simulink model "Slope_Road_SideSlipAngle_Vx_Estimation"  (R2024b)
settings: Solver=FixedStepAuto  StartTime=0.0  StopTime=7.5  FixedStep=0.001  RelTol=1e-4
values from neighbouring files (symbols this model uses):
  ax_long_1 = 1    [Init.m]
  ax_long_2 = 3    [Init.m]
  ax_long_3 = 6    [Init.m]
  ax_steer_1 = 0.5    [Init.m]
  ax_steer_2 = 1.5    [Init.m]
  ax_steer_3 = 3    [Init.m]
  ax_vx_thres1 = 0.5    [Init.m]
  ax_vx_thres2 = 3    [Init.m]
  Brush = [28.93,1.496,0.9486,0.06054]    [Init.m]
  delay_constant = 1/delay_length*ones(1,round(delay_length))    [Init.m]
  delta_thres = 3*3.14/180    (= 0.0523333333333)    [Init.m]
  deltarate_thres = 0.1    [Init.m]
  dg2rd = pi/180    (= 0.0174532925199)    [Init.m]
  excessive_wheel_intgr = 1000    [Init.m]
  filter_ratio_ax_ay = 0.2    [Init.m]
  g = 9.8    [Init.m]
  gao_ay = 1.5    [Init.m]
  gao_D_v = 0.2    [Init.m]
  gao_D_w = 0.03    [Init.m]
  gao_D_w1 = 0.25    [Init.m]
  gao_gz = 0.1    [Init.m]
  gao_Q = 1e-02    (= 0.01)    [Init.m]
  gao_R = 0.00077574*0.1    (= 7.7574e-05)    [Init.m]
  K_theta = 1    [Init.m]
  k_vx_vari_thres1 = 20    [Init.m]
  k_vx_vari_thres2 = 20    [Init.m]
  k_vx_vari_thres3 = 20    [Init.m]
  k_vy = 1/veh_m0    (= 0.000327653997379)    [Init.m]
  N_num = 6    [Init.m]
  para_long_1 = 1    [Init.m]
  para_long_2 = 100    [Init.m]
  para_long_3 = 100000000    [Init.m]
  para_long_4 = 100    [Init.m]
  para_steer_1 = 0.1    [Init.m]
  para_steer_2 = 10    [Init.m]
  para_steer_3 = 1000    [Init.m]
  para_steer_4 = 1000    [Init.m]
  rd2dg = 180/pi    (= 57.2957795131)    [Init.m]
  Steer_angle = 0    [Init.m]
  tao_1 = 6    [Init.m]
  time_interval = 1/Ts    (= 1000)    [Init.m]
  Ts = 0.001    [Init.m]
  u_init = 0.9    [Init.m]
  veh_bf = 1.600    (= 1.6)    [Init.m]
  veh_br = 1.740    (= 1.74)    [Init.m]
  veh_lf = 1.293    [Init.m]
  veh_lr = veh_l-veh_lf    (= 1.835)    [Init.m]
  veh_m0 = 3052    [Init.m]
  vx_cri = 1    [Init.m]
  vx_lowest = 0.01    [Init.m]
  vx_max_diff = 1    [Init.m]
  vy_new_ini = 0    [Init.m]
  wh_r = 0.346    [Init.m]
undefined symbols (not defined in the file or in its folder): DiscIntNeverNeededParam, front_gear_ratio, rear_gear_ratio, steer_ratio
libraries: simulink x7, Solver_SF x1
(part 2 of 2)

== system Slope_Road_SideSlipAngle_Vx_Estimation/vx estimation/detect overslip // excessive wheel slip(ews)/wheel acceleration deviation criterion/车轮加速度2/Subsystem1 ==
  In1 : Inport
  Mux : Mux  Inputs=10
  Unit Delay{1..9} (9 alike) : UnitDelay  SampleTime=-1  HasFrameUpgradeWarning=on
  last : Outport
  Out1 : Outport  Port=2
  wires:
  Mux/1 -> Out1/1
  In1/1 -> Mux/10, Unit Delay3/1
  Unit Delay9/1 -> last/1, Mux/1
  Unit Delay8/1 -> Mux/2, Unit Delay9/1
  Unit Delay7/1 -> Mux/3, Unit Delay8/1
  Unit Delay6/1 -> Mux/4, Unit Delay7/1
  Unit Delay5/1 -> Mux/5, Unit Delay6/1
  Unit Delay4/1 -> Mux/6, Unit Delay5/1
  Unit Delay1/1 -> Mux/8, Unit Delay2/1
  Unit Delay2/1 -> Mux/7, Unit Delay4/1
  Unit Delay3/1 -> Mux/9, Unit Delay1/1

== system Slope_Road_SideSlipAngle_Vx_Estimation/vx estimation/detect overslip // excessive wheel slip(ews)/wheel acceleration deviation criterion/车轮加速度2/Subsystem2 ==
  In1 : Inport
  Mux : Mux  Inputs=10
  Unit Delay{1..9} (9 alike) : UnitDelay  SampleTime=-1  HasFrameUpgradeWarning=on
  last : Outport
  Out1 : Outport  Port=2
  wires:
  Unit Delay3/1 -> Mux/9, Unit Delay1/1
  Unit Delay2/1 -> Mux/7, Unit Delay4/1
  Unit Delay1/1 -> Mux/8, Unit Delay2/1
  Unit Delay4/1 -> Mux/6, Unit Delay5/1
  Unit Delay5/1 -> Mux/5, Unit Delay6/1
  Unit Delay6/1 -> Mux/4, Unit Delay7/1
  Unit Delay7/1 -> Mux/3, Unit Delay8/1
  Unit Delay8/1 -> Mux/2, Unit Delay9/1
  Unit Delay9/1 -> Mux/1, last/1
  In1/1 -> Mux/10, Unit Delay3/1
  Mux/1 -> Out1/1

== system Slope_Road_SideSlipAngle_Vx_Estimation/vx estimation/detect overslip // excessive wheel slip(ews)/wheel acceleration deviation criterion/车轮加速度3/Subsystem ==
  In1 : Inport
  Mux : Mux  Inputs=10
  Unit Delay{,1..8} (9 alike) : UnitDelay  SampleTime=-1  HasFrameUpgradeWarning=on
  last : Outport
  Out1 : Outport  Port=2
  wires:
  Mux/1 -> Out1/1
  In1/1 -> Unit Delay/1, Mux/10
  Unit Delay8/1 -> last/1, Mux/1
  Unit Delay7/1 -> Unit Delay8/1, Mux/2
  Unit Delay6/1 -> Unit Delay7/1, Mux/3
  Unit Delay5/1 -> Unit Delay6/1, Mux/4
  Unit Delay4/1 -> Unit Delay5/1, Mux/5
  Unit Delay3/1 -> Unit Delay4/1, Mux/6
  Unit Delay1/1 -> Unit Delay2/1, Mux/8
  Unit Delay2/1 -> Unit Delay3/1, Mux/7
  Unit Delay/1 -> Unit Delay1/1, Mux/9

== system Slope_Road_SideSlipAngle_Vx_Estimation/vx estimation/detect overslip // excessive wheel slip(ews)/wheel acceleration deviation criterion/车轮加速度3/Subsystem1 ==
  In1 : Inport
  Mux : Mux  Inputs=10
  Unit Delay{1..9} (9 alike) : UnitDelay  SampleTime=-1  HasFrameUpgradeWarning=on
  last : Outport
  Out1 : Outport  Port=2
  wires:
  Unit Delay3/1 -> Unit Delay1/1, Mux/9
  Unit Delay2/1 -> Unit Delay4/1, Mux/7
  Unit Delay1/1 -> Unit Delay2/1, Mux/8
  Unit Delay4/1 -> Unit Delay5/1, Mux/6
  Unit Delay5/1 -> Unit Delay6/1, Mux/5
  Unit Delay6/1 -> Unit Delay7/1, Mux/4
  Unit Delay7/1 -> Unit Delay8/1, Mux/3
  Unit Delay8/1 -> Unit Delay9/1, Mux/2
  Unit Delay9/1 -> Mux/1, last/1
  In1/1 -> Unit Delay3/1, Mux/10
  Mux/1 -> Out1/1

== system Slope_Road_SideSlipAngle_Vx_Estimation/vx estimation/detect overslip // excessive wheel slip(ews)/wheel acceleration deviation criterion/车轮加速度3/Subsystem2 ==
  In1 : Inport
  Mux : Mux  Inputs=10
  Unit Delay{1..9} (9 alike) : UnitDelay  SampleTime=-1  HasFrameUpgradeWarning=on
  last : Outport
  Out1 : Outport  Port=2
  wires:
  Mux/1 -> Out1/1
  In1/1 -> Unit Delay3/1, Mux/10
  Unit Delay9/1 -> last/1, Mux/1
  Unit Delay8/1 -> Unit Delay9/1, Mux/2
  Unit Delay7/1 -> Unit Delay8/1, Mux/3
  Unit Delay6/1 -> Unit Delay7/1, Mux/4
  Unit Delay5/1 -> Unit Delay6/1, Mux/5
  Unit Delay4/1 -> Unit Delay5/1, Mux/6
  Unit Delay1/1 -> Unit Delay2/1, Mux/8
  Unit Delay2/1 -> Unit Delay4/1, Mux/7
  Unit Delay3/1 -> Unit Delay1/1, Mux/9

== system Slope_Road_SideSlipAngle_Vx_Estimation/vx estimation/detect overslip // excessive wheel slip(ews)/wheel acceleration deviation criterion/车轮加速度4/Subsystem ==
  In1 : Inport
  Mux : Mux  Inputs=10
  Unit Delay{,1..8} (9 alike) : UnitDelay  SampleTime=-1  HasFrameUpgradeWarning=on
  last : Outport
  Out1 : Outport  Port=2
  wires:
  Unit Delay/1 -> Mux/9, Unit Delay1/1
  Unit Delay2/1 -> Mux/7, Unit Delay3/1
  Unit Delay1/1 -> Mux/8, Unit Delay2/1
  Unit Delay3/1 -> Mux/6, Unit Delay4/1
  Unit Delay4/1 -> Mux/5, Unit Delay5/1
  Unit Delay5/1 -> Mux/4, Unit Delay6/1
  Unit Delay6/1 -> Mux/3, Unit Delay7/1
  Unit Delay7/1 -> Mux/2, Unit Delay8/1
  Unit Delay8/1 -> Mux/1, last/1
  In1/1 -> Mux/10, Unit Delay/1
  Mux/1 -> Out1/1

== system Slope_Road_SideSlipAngle_Vx_Estimation/vx estimation/detect overslip // excessive wheel slip(ews)/wheel acceleration deviation criterion/车轮加速度4/Subsystem1 ==
  In1 : Inport
  Mux : Mux  Inputs=10
  Unit Delay{1..9} (9 alike) : UnitDelay  SampleTime=-1  HasFrameUpgradeWarning=on
  last : Outport
  Out1 : Outport  Port=2
  wires:
  Mux/1 -> Out1/1
  In1/1 -> Mux/10, Unit Delay3/1
  Unit Delay9/1 -> last/1, Mux/1
  Unit Delay8/1 -> Mux/2, Unit Delay9/1
  Unit Delay7/1 -> Mux/3, Unit Delay8/1
  Unit Delay6/1 -> Mux/4, Unit Delay7/1
  Unit Delay5/1 -> Mux/5, Unit Delay6/1
  Unit Delay4/1 -> Mux/6, Unit Delay5/1
  Unit Delay1/1 -> Mux/8, Unit Delay2/1
  Unit Delay2/1 -> Mux/7, Unit Delay4/1
  Unit Delay3/1 -> Mux/9, Unit Delay1/1

== system Slope_Road_SideSlipAngle_Vx_Estimation/vx estimation/detect overslip // excessive wheel slip(ews)/wheel acceleration deviation criterion/车轮加速度4/Subsystem2 ==
  In1 : Inport
  Mux : Mux  Inputs=10
  Unit Delay{1..9} (9 alike) : UnitDelay  SampleTime=-1  HasFrameUpgradeWarning=on
  last : Outport
  Out1 : Outport  Port=2
  wires:
  Unit Delay3/1 -> Mux/9, Unit Delay1/1
  Unit Delay2/1 -> Mux/7, Unit Delay4/1
  Unit Delay1/1 -> Mux/8, Unit Delay2/1
  Unit Delay4/1 -> Mux/6, Unit Delay5/1
  Unit Delay5/1 -> Mux/5, Unit Delay6/1
  Unit Delay6/1 -> Mux/4, Unit Delay7/1
  Unit Delay7/1 -> Mux/3, Unit Delay8/1
  Unit Delay8/1 -> Mux/2, Unit Delay9/1
  Unit Delay9/1 -> Mux/1, last/1
  In1/1 -> Mux/10, Unit Delay3/1
  Mux/1 -> Out1/1

== matlab function Slope_Road_SideSlipAngle_Vx_Estimation/side slip angle estimation /side slip angle estimation/MATLAB Function ==
  data: delta input; m input; vx input; omega input; ay input; vy_hat_deri output; excita input; theta_hat input; fy_hat_star input; par_fystar_vy input; k_vy input; tao_1 input; Fx_front input; time_sig input; time_sig output; K_theta input; time_interval input; ema output; ota output
function [vy_hat_deri, time_sig,ema,ota] = fcn(delta, m, vx, omega, ay, excita, theta_hat, fy_hat_star,par_fystar_vy,k_vy, tao_1, Fx_front, time_sig, K_theta, time_interval)

if abs(m*ay)<abs(theta_hat*fy_hat_star) && par_fystar_vy>-abs(fy_hat_star)
    ema=-abs(fy_hat_star);
    ota=1/(2*max(abs(fy_hat_star),0.01));
else
    ema=par_fystar_vy;
    ota=1/max((ema^2+fy_hat_star^2)^(0.5),0.01);
end

%  vy_hat_deri=ay-omega*vx+k_vy*ota*ema*(m*ay-Fx_front*sin(delta)-theta_hat*fy_hat_star);  % 估计器公式
% vy_hat_deri=ay-omega*vx+k_vy*ota*ema*(m*ay-Fx_front*sin(delta)-fy_hat_star);  % 估计器公式
vy_hat_deri=ay-omega*vx+k_vy*ota*ema*(m*ay-fy_hat_star);  % 估计器公式



%  if excita==1  % 激励充足
% %      theta_hat_deri=tao_1*k_vy*ota*fy_hat_star*(m*ay-Fx_front*sin(delta)-theta_hat*fy_hat_star);  % 估计器公式
%      theta_hat_deri=tao_1*k_vy*ota*fy_hat_star*(m*ay-Fx_front*sin(delta)-fy_hat_star);  % 估计器公式
%      time_sig=0;
%  else          % 激励不足
%      time_sig=time_sig+1;
%      if time_sig>=time_interval    % 激励不足持续一段时间
%         theta_hat_deri=K_theta*(1-theta_hat) ;   % theta逐渐收敛到1
%      else
%         theta_hat_deri=0;     % theta不更新
%      end     
%  end

== matlab function Slope_Road_SideSlipAngle_Vx_Estimation/side slip angle estimation /MATLAB Function2 ==
  data: vx input; y output; vx_cri input
function y = fcn(vx,vx_cri)

if vx<=vx_cri
    y=vx_cri;
else
    y=vx;
end

== matlab function Slope_Road_SideSlipAngle_Vx_Estimation/vx estimation/Kalman-Filter/Kalman Gain/MATLAB Function ==
  data: ews input; R_update output; ax_pro input; vbest_believe input; gao_R input; gao_Q input; Q_update output; para_long_1 input; para_long_2 input; para_long_3 input; para_long_4 input; para_steer_1 input; para_steer_2 input; para_steer_3 input; para_steer_4 input; ax_long_1 input; ax_long_2 input; ax_long_3 input; ax_steer_1 input; ax_steer_2 input; ax_steer_3 input
function [R_update,Q_update] = fcn(ews, ax_pro, vbest_believe,gao_R,gao_Q,para_long_1,para_long_2,para_long_3,para_long_4,para_steer_1,para_steer_2,para_steer_3,para_steer_4,ax_long_1,ax_long_2,ax_long_3,ax_steer_1,ax_steer_2,ax_steer_3)
if  vbest_believe==0  % 没有侧向运动
   if ((sum(ews)>=0 & sum(ews)<=2) || abs(ax_pro)<=ax_long_1) && (abs(ax_pro)<=ax_long_2)
        R_update=para_long_1*gao_R;
        Q_update=gao_Q;
   elseif ((sum(ews)==3) || (abs(ax_pro)<=ax_long_2 & abs(ax_pro)>ax_long_1)) && (abs(ax_pro)<=ax_long_3)
        rate_long_1=(para_long_2-para_long_1)/(ax_long_2-ax_long_1);
        R_update=(para_long_1+rate_long_1*(abs(ax_pro)-ax_long_1))*gao_R;
        Q_update=gao_Q;
   else
        rate_long_2=(para_long_3-para_long_2)/(ax_long_3-ax_long_2);
        R_update=(para_long_2+rate_long_2*(abs(ax_pro)-ax_long_2))*gao_R;
        Q_update=para_long_4*gao_Q;
   end
else
   if (sum(ews)>=0 & sum(ews)<=2) || abs(ax_pro)<=ax_steer_1
        R_update=para_steer_1*gao_R;
        Q_update=gao_Q;
   elseif (sum(ews)==3) || (abs(ax_pro)<=ax_steer_2 & abs(ax_pro)>ax_steer_1)
        rate_steer_1=(para_steer_2-para_steer_1)/(ax_steer_2-ax_steer_1);
        R_update=(para_steer_1+rate_steer_1*(abs(ax_pro)-ax_steer_1))*gao_R;
        Q_update=gao_Q;
   else
        rate_steer_2=(para_steer_3-para_steer_2)/(ax_steer_3-ax_steer_2);
        R_update=(para_steer_2+rate_steer_2*(abs(ax_pro)-ax_steer_2))*gao_R;
        Q_update=para_steer_4*gao_Q;
   end
end

== matlab function Slope_Road_SideSlipAngle_Vx_Estimation/vx estimation/best wheel selection /MATLAB Function3 ==
  data: v output size=[1,1]; vrc input; ews input; ay input; gao_ay input; gz input; gao_gz input; Fxfl_sign input; Fxfr_sign input; Fxrl_sign input; Fxrr_sign input; v_best_believe output size=[1,1]; delta_rad input; deltarate_rads input; delta_thres input; deltarate_thres input
function [v,v_best_believe] = fcn(vrc,ews,ay,gao_ay,gz,gao_gz,Fxfl_sign,Fxfr_sign,Fxrl_sign,Fxrr_sign,delta_rad,deltarate_rads,delta_thres,deltarate_thres)


vFL = vrc(1);   % v_corr FL
vFR = vrc(2);   % v_corr FR
vRL = vrc(3);   % v_corr RL
vRR = vrc(4);   % v_corr RR
ewsFL = ews(1); % ews FL
ewsFR = ews(2); % ews FR
ewsRL = ews(3); % ews RL
ewsRR = ews(4); % ews RR
v=zeros(1,1);
v_choose_p=zeros(4,2);
v_choose_l=zeros(4,2);
v_choose = [ewsFL vFL Fxfl_sign; 
            ewsFR vFR Fxfr_sign; 
            ewsRL vRL Fxrl_sign; 
            ewsRR vRR Fxrr_sign]; % All velocities with corresponding EWS Flag
v_best_believe=boolean(1);

%我们发现，纵向加速度的测量值会受到坡度的影响，因此有时纵向加速度为正，实际车辆在减速，容易影响最优车速的选择；此外横摆角速度和侧向车速也会影响纵向加速度。因此我们采用每个车轮上是否有加速或减速意图（通过轮胎上施加的是驱动力还是制动力来判断）来判断某个轮胎处于驱动还是制动状态。
if ((abs(ay)>=gao_ay | abs(gz)>gao_gz | abs(delta_rad)>delta_thres | abs(deltarate_rads)>deltarate_thres) )  
    % 有侧向运动的情况
     if sum(ews(1:4)) == 4   % If all wheels have EWS, choose from all 4 wheels
        v_choose_f1 = [vFL Fxfl_sign; vFR Fxfr_sign; vRL Fxrl_sign; vRR Fxrr_sign];
        v=all_wheel_slip(v_choose_f1(:,1),sum(v_choose_f1(:,2)));
     else
        lenth_l=sum(v_choose(:,1)==0);  % 不打滑车轮数量
        num_index_l=(v_choose(:,1)==0);  % 车轮打滑为0，不打滑为1
        jj=0;
        for ii=1:4
            if num_index_l(ii)==1
                jj=jj+1;
                v_choose_l(jj,:)=v_choose(ii,2:3);  % 筛选不打滑车轮的信息
            end
        end
        if lenth_l==4  % 四轮不打滑
             v=all_wheel_slip_lat(v_choose_l(1:lenth_l,1),lenth_l);
        elseif lenth_l==3  % 三轮不打滑
             v=all_wheel_slip_lat(v_choose_l(1:lenth_l,1),lenth_l);
        else
             v=mean(v_choose_l(1:lenth_l,1));
        end
    end
    v_best_believe=boolean(1);
else
    if sum(ews(1:4)) == 4   % If all wheels have EWS, choose from all 4 wheels
        v_choose_f2 = [vFL Fxfl_sign; vFR Fxfr_sign; vRL Fxrl_sign; vRR Fxrr_sign];
        v=all_wheel_slip(v_choose_f2(:,1),sum(v_choose_f2(:,2)));  %取最小或最大轮速
    else
        lenth=sum(v_choose(:,1)==0);
        num_index=(v_choose(:,1)==0);
        j=0;
        for i=1:4
            if num_index(i)==1
                j=j+1;
                v_choose_p(j,:)=v_choose(i,2:3);  % 筛选不打滑车轮的信息
            end
        end
        if (sum(v_choose_p(:,2)>0)==lenth)  % 不打滑车轮的纵向力均为正
           v=min(v_choose_p(1:lenth,1));
        elseif (sum(v_choose_p(:,2)<0)==lenth)  % 不打滑车轮的纵向力均为负
           v=max(v_choose_p(1:lenth,1)); 
        else   % 不打滑车轮的纵向力正负不统一
           v=all_wheel_slip_long(v_choose_p(:,1),lenth);  
        end
    end
  v_best_believe=boolean(0);
end
end

== matlab function Slope_Road_SideSlipAngle_Vx_Estimation/vx estimation/detect overslip // excessive wheel slip(ews)/MATLAB Function ==
  data: u1 input; y output; u2 input; vr input; excessive_wheel_intgr input; intgr_num_pre input; intgr_num output; vx_max_diff input
function [y, intgr_num] = fcn(u1,u2,vr,excessive_wheel_intgr,intgr_num_pre,vx_max_diff)

num=length(u2);
y=zeros(num,1);
vx_ave=mean(vr);
vx_diff=max(abs(vr-vx_ave));
intgr_num=zeros(num,1);
for i=1:num
    if u1(i)>=1 
        y(i)=u1(i)+u2(i);
        intgr_num(i)=0;
    elseif u1(i)<1 & intgr_num_pre(i)<=excessive_wheel_intgr(i)
        if vx_diff>=vx_max_diff
            y(i)=u1(i)+u2(i);
            intgr_num(i)=0;
        else
            y(i)=u1(i)+u2(i);
            intgr_num(i)=intgr_num_pre(i)+1;  % 若u1=0，四轮轮速差异不大，计时1s（或0.1s），在1s内信任u2，1s后不信任u2
        end
    else
        y(i)=u1(i);%+u2(i);
        intgr_num(i)=0;
    end
end

== matlab function Slope_Road_SideSlipAngle_Vx_Estimation/vx estimation/detect overslip // excessive wheel slip(ews)/pre estimation deviation criterion/Embedded MATLAB Function ==
  data: u input; y output; gao_D_v input
function y = fcn(u,gao_D_v)
%#eml



p=size(u);
if p(1)~=4 | p(2)~=1
    y=zeros(4,1);
    y=gao_D_v+0.01;
else
         y=u;
end

== matlab function Slope_Road_SideSlipAngle_Vx_Estimation/vx estimation/detect overslip // excessive wheel slip(ews)/wheel acceleration deviation criterion/Embedded MATLAB Function ==
  data: u input; y output; gao_D_w1 input; p output
function [y,p] = fcn(u,gao_D_w1)
%#eml

p=size(u);
if p(1)~=4 | p(2)~=1
    y=zeros(4,1);
    y=gao_D_w1+0.01;
else
         y=u;

end

== matlab function Slope_Road_SideSlipAngle_Vx_Estimation/vx estimation/detect overslip // excessive wheel slip(ews)/wheel acceleration deviation criterion/车轮加速度1/Embedded MATLAB Function ==
  data: y input; a output; N input
function a = fcn(y, N)
%#eml
ak=single(0);
 k=single(length(y));
for n=0:N-1
h= 6/(N*(N+1))*(1-2*n/(N-1));
ak=ak+h*y(k-n);
end
a = ak;

== matlab function Slope_Road_SideSlipAngle_Vx_Estimation/vx estimation/detect overslip // excessive wheel slip(ews)/wheel acceleration deviation criterion/车轮加速度2/Embedded MATLAB Function ==
  data: y input; a output; N input; m output
function [a,m] = fcn(y, N)
%#eml
ak=single(0);
 k=single(length(y));
for n=0:N-1
h= 6/(N*(N+1))*(1-2*n/(N-1));
ak=ak+h*y(k-n);
end
a = ak;
m=length(y);

== matlab function Slope_Road_SideSlipAngle_Vx_Estimation/vx estimation/detect overslip // excessive wheel slip(ews)/wheel acceleration deviation criterion/车轮加速度3/Embedded MATLAB Function ==
  data: y input; a output; N input
function a = fcn(y, N)
%#eml
ak=single(0);
 k=single(length(y));
for n=0:N-1
h= 6/(N*(N+1))*(1-2*n/(N-1));
ak=ak+h*y(k-n);
end
a = ak;

== matlab function Slope_Road_SideSlipAngle_Vx_Estimation/vx estimation/detect overslip // excessive wheel slip(ews)/wheel acceleration deviation criterion/车轮加速度4/Embedded MATLAB Function ==
  data: y input; a output; N input
function a = fcn(y, N)
%#eml
ak=single(0);
 k=single(length(y));
for n=0:N-1
h= 6/(N*(N+1))*(1-2*n/(N-1));
ak=ak+h*y(k-n);
end
a = ak;

== matlab function Slope_Road_SideSlipAngle_Vx_Estimation/vx estimation/detect overslip // excessive wheel slip(ews)/wheel speed change criterion/Embedded MATLAB Function ==
  data: u input; y output; gao_D_w input
function y = fcn(u,gao_D_w)
%#eml
p=size(u);
if p(1)~=4 | p(2)~=1
    y=zeros(4,1);
    y=gao_D_w+0.01;
else
         y=u;
end

== matlab function Slope_Road_SideSlipAngle_Vx_Estimation/vx estimation/front_rear_drive process/Atomic Subsystem/MATLAB Function ==
  data: ax input; y output; ax_vx_thres1 input; ax_vx_thres2 input; k_vx_vari_thres1 input; k_vx_vari_thres2 input; k_vx_vari_thres3 input
function y = fcn(ax,ax_vx_thres1,ax_vx_thres2,k_vx_vari_thres1,k_vx_vari_thres2,k_vx_vari_thres3)
if abs(ax)<=ax_vx_thres1
    y=k_vx_vari_thres1;
elseif abs(ax)>ax_vx_thres1 & abs(ax)<=ax_vx_thres2
     y=k_vx_vari_thres2;
else
y=k_vx_vari_thres3;
end

== matlab function Slope_Road_SideSlipAngle_Vx_Estimation/vx estimation/wheel speed correction to CoG/轮速到质心处车速 ==
  data: u input; v_rCoG output size=[4 1]; v input; delta_rad input; lf input; yawrate_rads input
function v_rCoG = fcn(u,v,delta_rad,lf,yawrate_rads)
v_rCoG=zeros(4,1);
% v_rCoG(1)=(u(1)-(lf*yawrate_rads+vy_ms_esti)*sin(delta_rad))/cos(delta_rad)+v(1);
% v_rCoG(2)=(u(2)-(lf*yawrate_rads+vy_ms_esti)*sin(delta_rad))/cos(delta_rad)+v(2);
v_rCoG(1)=u(1)+v(1);
v_rCoG(2)=u(2)+v(2);
v_rCoG(3)=u(3)+v(3);
v_rCoG(4)=u(4)+v(4);

== matlab function Slope_Road_SideSlipAngle_Vx_Estimation/vx estimation/倒挡车速计算/MATLAB Function ==
  data: vx_rear output; v_rCoG input; wheel_torque input; rear_drive_enable input
function vx_rear = fcn(v_rCoG,wheel_torque,rear_drive_enable)
if wheel_torque(1)>=0
    torque_sign_fl=1;
else
    torque_sign_fl=-1;
end
if wheel_torque(2)>=0
    torque_sign_fr=1;
else
    torque_sign_fr=-1;
end
if wheel_torque(3)>=0
    torque_sign_rl=1;
else
    torque_sign_rl=-1;
end
if wheel_torque(4)>=0
    torque_sign_rr=1;
else
    torque_sign_rr=-1;
end

if torque_sign_fl+torque_sign_fr+torque_sign_rl+torque_sign_rr>=2
    vx_rear=max(abs(v_rCoG)); %倒车时如果电机力矩为正，说明在倒车时减速，取四个轮速中最大的车速
else
    vx_rear=min(abs(v_rCoG));%倒车时如果电机力矩为负，说明在倒车时加速或匀速，取四个轮速中最小的为车速
end
if rear_drive_enable==1
vx_rear=-vx_rear;
else
vx_rear=vx_rear;
end

== matlab function Slope_Road_SideSlipAngle_Vx_Estimation/side slip angle estimation /side slip angle estimation/MATLAB Function2 ==
  data: k input; vy output; vy_kin input; vy_dyn input; theta input; k output
function [vy, k] = fcn(k, vy_kin, vy_dyn, theta)
if abs(theta-0.6)<0.001
    k = min(k*1.5,0.9);
end
vy = vy_kin*k+vy_dyn*(1-k);

== matlab function Slope_Road_SideSlipAngle_Vx_Estimation/side slip angle estimation /side slip angle estimation/MATLAB Function1 ==
  data: delta0 input; delta input; lf input; lr input; bf input; br input; a input; b input; c input; d input; vx0 input; omega0 input; fy_hat_star output; par_fystar_vy output; Fz_fl input; Fz_fr input; Fz_rl input; Fz_rr input; Fxf input; vy_hat input; Fyf output; Fyr output; k input; alpha_f output; alpha_r output; theta input
function [fy_hat_star,par_fystar_vy,Fyf,Fyr,alpha_f,alpha_r] = fcn(delta0,delta,lf,lr,bf,br,a,b,c,d,vx0,omega0,Fz_fl,Fz_fr,Fz_rl,Fz_rr,Fxf,vy_hat,k,theta)

if theta<0.5
    k = k*1.2;
elseif theta<0.85
    k = k*1.08;
end
% theta = 0.4;
[Fyf0,Fyr0,pderi_Fyf_vy,pderi_Fyr_vy,alpha_f,alpha_r] = Fyf_Fyr_cal_new(theta,lf,lr,bf,br,a,b,c,d,vx0,omega0,delta0,vy_hat,Fz_fl,Fz_fr,Fz_rl,Fz_rr);

if abs(Fyf0)>1
    Fyf = Fyf0/k; % 0.1m/s-1.27, 0.2m/s-1.20, 1.2m/s-1.20
else
    Fyf = 0;
end
if abs(Fyr0)>1
    Fyr = Fyr0/k;  % 0.1m/s-1.27, 0.2m/s-1.20, 1.2m/s-1.20
else
    Fyr = 0;
end

fy_hat_star = Fyf*cos(delta)+Fyr+Fxf*sin(delta);
par_fystar_vy=pderi_Fyf_vy+pderi_Fyr_vy;
if abs(par_fystar_vy)>1
    par_fystar_vy = par_fystar_vy;
else
    par_fystar_vy = -400000;
end
